simulink model "RonStatic_Fig10"  (R2022b)
settings: Solver=FixedStepDiscrete  StartTime=0.0  StopTime=468  FixedStep=1  RelTol=1e-3
model workspace (MAT data in the model file):
  staticInput = [0 1 2 3 4 5 6 7 8 9 10 11 ... (1407 elements, 469x3)]
settings Model: Creator=Greatlovers  LastModifiedBy=Greatlovers
settings DataIOCC: ExternalInput=getVariable(get_param('RonStatic_Fig10','ModelWorkspace'),'staticInput')  LoadExternalInput=on  OutputSaveName=staticY

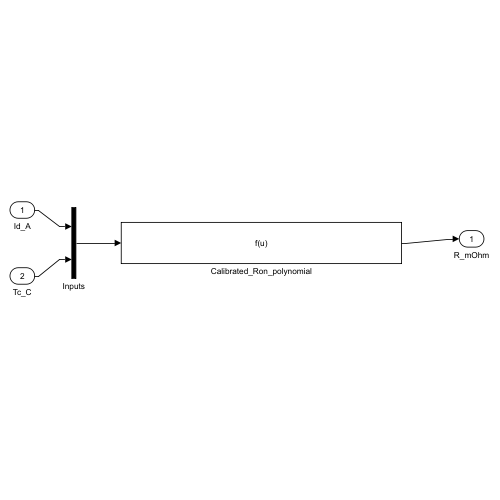
[thumbnail: Simulink's stored preview of the top-level diagram]
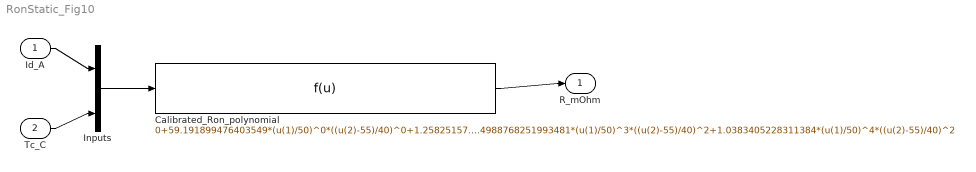
== system RonStatic_Fig10 ==
  Id_A : Inport
  Tc_C : Inport  Port=2
  Calibrated_Ron_polynomial : Fcn  Expr=0+59.191899476403549*(u(1)/50)^0*((u(2)-55)/40)^0+1.2582515710920177*(u(1)/50)^1*((u(2)-55)/40)^0+0.61381375818996953*(u(1)/50)^2*((u(2)-55)/40)^0+-0.92127083590050085*(u(1)/50)^3*((u(2)-55)/40)^0+3.8653416481657192*(u(1)/50)^4*((u(2)-55)/40)^0+16.650381489503793*(u(1)/50)^0*((u(2)-55)/40)^1+-0.29309342495435298*(u(1)/50)^1*((u(2)-55)/40)^1+-1.5875159190221082*(u(1)/50)^2*((u(2)-55)/40)^1+0.14310637913834642*(u(1)/50)^3*((u(2)-55)/40)^1+3.9748760177435076*(u(1)/50)^4*((u(2)-55)/40)^1+0.75480348874822401*(u(1)/50)^0*((u(2)-55)/40)^2+-0.38568150293168052*(u(1)/50)^1*((u(2)-55)/40)^2+0.16030076037665938*(u(1)/50)^2*((u(2)-55)/40)^2+1.4988768251993481*(u(1)/50)^3*((u(2)-55)/40)^2+1.0383405228311384*(u(1)/50)^4*((u(2)-55)/40)^2
  Inputs : Mux  Inputs=2
  R_mOhm : Outport
  wires:
  Id_A/1 -> Inputs/1
  Tc_C/1 -> Inputs/2
  Inputs/1 -> Calibrated_Ron_polynomial/1
  Calibrated_Ron_polynomial/1 -> R_mOhm/1
